simulink model "snap_adc5g_spec_rpi"  (R2019a)
settings: Solver=VariableStepDiscrete  StartTime=0.0  StopTime=10.0  RelTol=1e-3
undefined symbols (not defined in the file): pfb_coeff_gen_calc
libraries: xbsIndex_r4 x13965, casper_library_misc x80, casper_library_delays x43, xps_library x5, xbsReplacements_r4 x2, casper_library_communications x1
(part 7 of 152)

== system snap_adc5g_spec_rpi/fft_wideband_real/fft_direct ==
  sync : Inport
  shift : Inport  Port=2
  in00 : Inport  Port=3
  in01 : Inport  Port=4
  in02 : Inport  Port=5
  in03 : Inport  Port=6
  in10 : Inport  Port=7
  in11 : Inport  Port=8
  in12 : Inport  Port=9
  in13 : Inport  Port=10
  abus : Subsystem  AncestorBlock=casper_library_flow_control/bus_create  mask(bus_create){inputNum=4}
      mask prompts: inputNum "Number of inputs:"
      mask init:
      | bus_create_init(gcb,...
      |     'inputNum', inputNum);
  adebus0_0 : Subsystem  AncestorBlock=casper_library_flow_control/bus_expand  mask(bus_expand){mode=divisions of equal size, outputNum=2, outputWidth=[72 72], outputBinaryPt=[0 0], outputArithmeticType=[0 0], show_format=off, outputToWorkspace=off, variablePrefix=out, outputToModelAsWell=on}
      mask prompts: outputNum "Number of outputs:"; outputWidth "Output width:"; outputBinaryPt "Output binary point position:"; outputArithmeticType "Output arithmetic type (ufix=0, fix=1, bool=2):"; show_format "Print format string?"; outputToWorkspace "Output to workspace?"; variablePrefix "Variable name prefix:"; outputToModelAsWell "Output to model as well?"
      mask help:
      | Expands a 'bus' made using a bus_create or Xilinx
      | concat block.
      | The input will be divided into the specified number
      | of outputs with the specified arithmetic types.
      | Divisions are made from most significant bit.
      mask init: same as snap_adc5g_spec_rpi/ss_adc/ctrl_split
      settings: AttributesFormatString=2 outputs
      mask TypeOptions mode: divisions of equal size | divisions of arbitrary size
      mask Callback mode: bus_expand_callback();
      mask Callback outputWidth: bus_expand_callback();
      mask Callback outputToWorkspace: bus_expand_callback();
  adebus1_0 : Subsystem  AncestorBlock=casper_library_flow_control/bus_expand  mask(bus_expand){mode=divisions of equal size, outputNum=2, outputWidth=[36 36], outputBinaryPt=[0 0], outputArithmeticType=[0 0], show_format=off, outputToWorkspace=off, variablePrefix=out, outputToModelAsWell=on}
      mask prompts: outputNum "Number of outputs:"; outputWidth "Output width:"; outputBinaryPt "Output binary point position:"; outputArithmeticType "Output arithmetic type (ufix=0, fix=1, bool=2):"; show_format "Print format string?"; outputToWorkspace "Output to workspace?"; variablePrefix "Variable name prefix:"; outputToModelAsWell "Output to model as well?"
      mask help:
      | Expands a 'bus' made using a bus_create or Xilinx
      | concat block.
      | The input will be divided into the specified number
      | of outputs with the specified arithmetic types.
      | Divisions are made from most significant bit.
      mask init: same as snap_adc5g_spec_rpi/ss_adc/ctrl_split
      settings: AttributesFormatString=2 outputs
      mask TypeOptions mode: divisions of equal size | divisions of arbitrary size
      mask Callback mode: bus_expand_callback();
      mask Callback outputWidth: bus_expand_callback();
      mask Callback outputToWorkspace: bus_expand_callback();
  adebus1_1 : Subsystem  AncestorBlock=casper_library_flow_control/bus_expand  mask(bus_expand){mode=divisions of equal size, outputNum=2, outputWidth=[36 36], outputBinaryPt=[0 0], outputArithmeticType=[0 0], show_format=off, outputToWorkspace=off, variablePrefix=out, outputToModelAsWell=on}
      mask prompts: outputNum "Number of outputs:"; outputWidth "Output width:"; outputBinaryPt "Output binary point position:"; outputArithmeticType "Output arithmetic type (ufix=0, fix=1, bool=2):"; show_format "Print format string?"; outputToWorkspace "Output to workspace?"; variablePrefix "Variable name prefix:"; outputToModelAsWell "Output to model as well?"
      mask help:
      | Expands a 'bus' made using a bus_create or Xilinx
      | concat block.
      | The input will be divided into the specified number
      | of outputs with the specified arithmetic types.
      | Divisions are made from most significant bit.
      mask init: same as snap_adc5g_spec_rpi/ss_adc/ctrl_split
      settings: AttributesFormatString=2 outputs
      mask TypeOptions mode: divisions of equal size | divisions of arbitrary size
      mask Callback mode: bus_expand_callback();
      mask Callback outputWidth: bus_expand_callback();
      mask Callback outputToWorkspace: bus_expand_callback();
  bbus : Subsystem  AncestorBlock=casper_library_flow_control/bus_create  mask(bus_create){inputNum=4}
      mask prompts: inputNum "Number of inputs:"
      mask init:
      | bus_create_init(gcb,...
      |     'inputNum', inputNum);
  bdebus0_0 : Subsystem  AncestorBlock=casper_library_flow_control/bus_expand  mask(bus_expand){mode=divisions of equal size, outputNum=2, outputWidth=[72 72], outputBinaryPt=[0 0], outputArithmeticType=[0 0], show_format=off, outputToWorkspace=off, variablePrefix=out, outputToModelAsWell=on}
      mask prompts: outputNum "Number of outputs:"; outputWidth "Output width:"; outputBinaryPt "Output binary point position:"; outputArithmeticType "Output arithmetic type (ufix=0, fix=1, bool=2):"; show_format "Print format string?"; outputToWorkspace "Output to workspace?"; variablePrefix "Variable name prefix:"; outputToModelAsWell "Output to model as well?"
      mask help:
      | Expands a 'bus' made using a bus_create or Xilinx
      | concat block.
      | The input will be divided into the specified number
      | of outputs with the specified arithmetic types.
      | Divisions are made from most significant bit.
      mask init: same as snap_adc5g_spec_rpi/ss_adc/ctrl_split
      settings: AttributesFormatString=2 outputs
      mask TypeOptions mode: divisions of equal size | divisions of arbitrary size
      mask Callback mode: bus_expand_callback();
      mask Callback outputWidth: bus_expand_callback();
      mask Callback outputToWorkspace: bus_expand_callback();
  bdebus1_0 : Subsystem  AncestorBlock=casper_library_flow_control/bus_expand  mask(bus_expand){mode=divisions of equal size, outputNum=2, outputWidth=[36 36], outputBinaryPt=[0 0], outputArithmeticType=[0 0], show_format=off, outputToWorkspace=off, variablePrefix=out, outputToModelAsWell=on}
      mask prompts: outputNum "Number of outputs:"; outputWidth "Output width:"; outputBinaryPt "Output binary point position:"; outputArithmeticType "Output arithmetic type (ufix=0, fix=1, bool=2):"; show_format "Print format string?"; outputToWorkspace "Output to workspace?"; variablePrefix "Variable name prefix:"; outputToModelAsWell "Output to model as well?"
      mask help:
      | Expands a 'bus' made using a bus_create or Xilinx
      | concat block.
      | The input will be divided into the specified number
      | of outputs with the specified arithmetic types.
      | Divisions are made from most significant bit.
      mask init: same as snap_adc5g_spec_rpi/ss_adc/ctrl_split
      settings: AttributesFormatString=2 outputs
      mask TypeOptions mode: divisions of equal size | divisions of arbitrary size
      mask Callback mode: bus_expand_callback();
      mask Callback outputWidth: bus_expand_callback();
      mask Callback outputToWorkspace: bus_expand_callback();
  bdebus1_1 : Subsystem  AncestorBlock=casper_library_flow_control/bus_expand  mask(bus_expand){mode=divisions of equal size, outputNum=2, outputWidth=[36 36], outputBinaryPt=[0 0], outputArithmeticType=[0 0], show_format=off, outputToWorkspace=off, variablePrefix=out, outputToModelAsWell=on}
      mask prompts: outputNum "Number of outputs:"; outputWidth "Output width:"; outputBinaryPt "Output binary point position:"; outputArithmeticType "Output arithmetic type (ufix=0, fix=1, bool=2):"; show_format "Print format string?"; outputToWorkspace "Output to workspace?"; variablePrefix "Variable name prefix:"; outputToModelAsWell "Output to model as well?"
      mask help:
      | Expands a 'bus' made using a bus_create or Xilinx
      | concat block.
      | The input will be divided into the specified number
      | of outputs with the specified arithmetic types.
      | Divisions are made from most significant bit.
      mask init: same as snap_adc5g_spec_rpi/ss_adc/ctrl_split
      settings: AttributesFormatString=2 outputs
      mask TypeOptions mode: divisions of equal size | divisions of arbitrary size
      mask Callback mode: bus_expand_callback();
      mask Callback outputWidth: bus_expand_callback();
      mask Callback outputToWorkspace: bus_expand_callback();
  butterfly0_0 : Subsystem  AncestorBlock=casper_library_ffts/butterfly_direct  mask(butterfly_direct){n_inputs=4, biplex=off, FFTSize=13, Coeffs=[ 0 1024 512 1536 256 1280 768 1792 128 1152 640 1664 384 1408 896 1920 64 1088 576 1600 320 1344 832 1856 192 1216 704 1728 448 1472 960 1984 32 1056 544 1568 288 1312 800 1824 160 1184 672 1696 416 1440 928 1952 96 1120 608 1632 352 1376 864 1888 224 1248 736 1760 480 1504 992 2016 16 1040 528 1552 272 1296 784 1808 144 1168 656 1680 400 1424 912 1936 80 1104 592 1616 336 1360 848 1872 208 1232 720 1744 464 1488 976 2000 48 1072 560 1584 304 1328 816 1840 176 1200 688 1712 432 1456 944 1968 112 1136 624 1648 368 1392 880 1904 240 1264 752 1776 496 1520 1008 2032 8 1032 520 1544 264 1288 776 1800 136 1160 648 1672 392 1416 904 1928 72 1096 584 1608 328 1352 840 1864 200 1224 712 1736 456 1480 968 1992 40 1064 552 1576 296 1320 808 1832 168 1192 680 1704 424 1448 936 1960 104 1128 616 1640 360 1384 872 1896 232 1256 744 1768 488 1512 1000 2024 24 1048 536 1560 280 1304 792 1816 152 1176 664 1688 408 1432 920 1944 88 1112 600 1624 344 1368 856 1880 216 1240 728 1752 472 1496 984 2008 56 1080 568 1592 312 1336 824 1848 184 1208 696 1720 440 1464 952 1976 120 1144 632 1656 376 1400 888 1912 248 1272 760 1784 504 1528 1016 2040 4 1028 516 1540 260 1284 772 1796 132 1156 644 1668 388 1412 900 1924 68 1092 580 1604 324 1348 836 1860 196 1220 708 1732 452 1476 964 1988 36 1060 548 1572 292 1316 804 1828 164 1188 676 1700 420 1444 932 1956 100 1124 612 1636 356 1380 868 1892 228 1252 740 1764 484 1508 996 2020 20 1044 532 1556 276 1300 788 1812 148 1172 660 1684 404 1428 916 1940 84 1108 596 1620 340 1364 852 1876 212 1236 724 1748 468 1492 980 2004 52 1076 564 1588 308 1332 820 1844 180 1204 692 1716 436 1460 948 1972 116 1140 628 1652 372 1396 884 1908 244 1268 756 1780 500 1524 1012 2036 12 1036 524 1548 268 1292 780 1804 140 1164 652 1676 396 1420 908 1932 76 1100 588 1612 332 1356 844 1868 204 1228 716 1740 460 1484 972 1996 44 1068 556 1580 300 1324 812 1836 172 1196 684 1708 428 1452 940 1964 108 1132 620 1644 364 1388 876 1900 236 1260 748 1772 492 1516 1004 2028 28 1052 540 1564 284 1308 796 1820 156 1180 668 1692 412 1436 924 1948 92 1116 604 1628 348 1372 860 1884 220 1244 732 1756 476 1500 988 2012 60 1084 572 1596 316 1340 828 1852 188 1212 700 1724 444 1468 956 1980 124 1148 636 1660 380 1404 892 1916 252 1276 764 1788 508 1532 1020 2044 2 1026 514 1538 258 1282 770 1794 130 1154 642 1666 386 1410 898 1922 66 1090 578 1602 322 1346 834 1858 194 1218 706 1730 450 1474 962 1986 34 1058 546 1570 290 1314 802 1826 162 1186 674 1698 418 1442 930 1954 98 1122 610 1634 354 1378 866 1890 226 1250 738 1762 482 1506 994 2018 18 1042 530 1554 274 1298 786 1810 146 1170 658 1682 402 1426 914 1938 82 1106 594 1618 338 1362 850 1874 210 1234 722 1746 466 1490 978 2002 50 1074 562 1586 306 1330 818 1842 178 1202 690 1714 434 1458 946 1970 114 1138 626 1650 370 1394 882 1906 242 1266 754 1778 498 1522 1010 2034 10 1034 522 1546 266 1290 778 1802 138 1162 650 1674 394 1418 906 1930 74 1098 586 1610 330 1354 842 1866 202 1226 714 1738 458 1482 970 1994 42 1066 554 1578 298 1322 810 1834 170 1194 682 1706 426 1450 938 1962 106 1130 618 1642 362 1386 874 1898 234 1258 746 1770 490 1514 1002 2026 26 1050 538 1562 282 1306 794 1818 154 1178 666 1690 410 1434 922 1946 90 1114 602 1626 346 1370 858 1882 218 1242 730 1754 474 1498 986 2010 58 1082 570 1594 314 1338 826 1850 186 1210 698 1722 442 1466 954 1978 122 1146 634 1658 378 1402 890 1914 250 1274 762 1786 506 1530 1018 2042 6 1030 518 1542 262 1286 774 1798 134 1158 646 1670 390 1414 902 1926 70 1094 582 1606 326 1350 838 1862 198 1222 710 1734 454 1478 966 1990 38 1062 550 1574 294 1318 806 1830 166 1190 678 1702 422 1446 934 1958 102 1126 614 1638 358 1382 870 1894 230 1254 742 1766 486 1510 998 2022 22 1046 534 1558 278 1302 790 1814 150 1174 662 1686 406 1430 918 1942 86 1110 598 1622 342 1366 854 1878 214 1238 726 1750 470 1494 982 2006 54 1078 566 1590 310 1334 822 1846 182 1206 694 1718 438 1462 950 1974 118 1142 630 1654 374 1398 886 1910 246 1270 758 1782 502 1526 1014 2038 14 ...(+5134 chars)], StepPeriod=0, coeff_bit_width=18, input_bit_width=18, bin_pt_in=17, downshift=off, async=off, floating_point=off, float_type=single, exp_width=8, frac_width=24, add_latency=1, mult_latency=2, bram_latency=3, conv_latency=1, add_pipe_latency=0, mult_pipe_latency=0, quantization=Round  (unbiased: Even Values), overflow=Wrap, coeffs_bit_limit=9, coeff_sharing=on, coeff_decimation=on, coeff_generation=off, cal_bits=1, n_bits_rotation=25, max_fanout=4, use_hdl=on, use_embedded=off, bitgrowth=off, hardcode_shifts=off, dsp48_adders=off}
      mask prompts: n_inputs "number inputs"; biplex "Used in biplex FFT"; FFTSize "Size of FFT: (2^? pts)"; Coeffs "Coefficients: (0 to 2^(FFTSize-1)-1)"; StepPeriod "Coefficient Step Period: (2^?)"; coeff_bit_width "Coefficient Bit Width"; input_bit_width "Input Bit Width"; bin_pt_in "Input binary point"; async "asynchronous operation"; floating_point "floating point"; float_type "float type"; exp_width "exponent width"; frac_width "fraction width"; add_latency "Add Latency"; mult_latency "Mult Latency"; bram_latency "BRAM Latency"; conv_latency "Convert latency"; add_pipe_latency "Add Pipeline Latency"; mult_pipe_latency "Mult Pipeline Latency"; quantization "Quantization Behavior"; overflow "Overflow Behavior"; coeffs_bit_limit "Number bits above which to store stage's coefficients in BRAM (2^? bits)"; coeff_sharing "BRAM sharing in coeff storage"; coeff_decimation "Store a fraction of coeff factors where useful"; coeff_generation "Generate coeffs with multipliers where useful"; cal_bits "Number calibration locations when generating coeffs (2^?)"; n_bits_rotation "Feedback rotation vector resolution"; max_fanout "Maximum fanout"; use_hdl "Use behavioural HDL for multipliers"; use_embedded "Use embedded multipliers"; bitgrowth "Bit growth instead of shifting"; hardcode_shifts "Hardcode shift schedule"; dsp48_adders "Use DSP48s for adders"
      mask help: FFT internal block.
      mask init:
      | butterfly_direct_init(gcb, ...
      |    'n_inputs', n_inputs, ...
      |    'biplex', biplex, ...
      |    'FFTSize', FFTSize, ...
      |    'Coeffs', Coeffs, ...
      |    'StepPeriod', StepPeriod, ...
      |    'coeff_bit_width', coeff_bit_width, ...
      |    'input_bit_width', input_bit_width, ...
      |    'bin_pt_in', bin_pt_in, ...
      |    'hardcode_shifts', hardcode_shifts, ...
      |    'bitgrowth', bitgrowth, ...
      |    'downshift', downshift, ...
      |    'floating_point', floating_point, ...
      |    'float_type', float_type, ...
      |    'exp_width', exp_width, ...
      |    'frac_width', frac_width, ...   
      |    'async', async, ...
      |    'add_latency', add_latency, ...
      |    'mult_latency', mult_latency, ...
      |    'bram_latency', bram_latency, ...
      |    'conv_latency', conv_latency, ...
      |    'add_pipe_latency', add_pipe_latency, ...
      |    'mult_pipe_latency', mult_pipe_latency, ...        
      |    'quantization', quantization, ...
      |    'overflow', overflow, ...
      |    'coeffs_bit_limit', coeffs_bit_limit, ...    
      |    'coeff_sharing', coeff_sharing, ...
      |    'coeff_decimation', coeff_decimation, ...
      |    'coeff_generation', coeff_generation, ...
      |    'cal_bits', cal_bits, ...
      |    'n_bits_rotation', n_bits_rotation, ...
      |    'max_fanout', max_fanout, ...
      |    'use_hdl', use_hdl, ...
      |    'use_embedded', use_embedded, ...
      |    'dsp48_adders', dsp48_adders);
      settings: AttributesFormatString=twiddle_general
      mask Callback floating_point:
      | onoff = get_param(gcb, 'floating_point');
      | if strcmp(onoff,'on')
      |     enable_fixpt = 'off'
      |     set_param_state(gcb, 'float_type', 'on')
      | 
      |     f_type = get_param(gcb, 'float_type')
      |     if strcmp(f_type,'custom')
      |         set_param_state(gcb, 'exp_width', 'on')
      |         set_param_state(gcb, 'frac_width', 'on')
      |     else
      |         set_param_state(gcb, 'exp_width', 'off')
      |         set_param_state(gcb, 'frac_width', 'off')
      |     end
      | 
      | 
      | else
      |     enable_fixpt = 'on'
      |     set_param_state(gcb, 'float_type', 'off')
      |     set_param_state(gcb, 'exp_width', 'off')
      |     set_param_state(gcb, 'frac_width', 'off')
      | end
      | 
      | set_param_state(gcb, 'input_bit_width', enable_fixpt)
      | set_param_state(gcb, 'bin_pt_in', enable_fixpt)
      | set_param_state(gcb, 'coeff_bit_width', enable_fixpt)
      mask TypeOptions float_type: single | custom
      mask Callback float_type:
      | f_type = get_param(gcb, 'float_type')
      | if strcmp(f_type,'custom')
      |     set_param_state(gcb, 'exp_width', 'on')
      |     set_param_state(gcb, 'frac_width', 'on')
      | else
      |     set_param_state(gcb, 'exp_width', 'off')
      |     set_param_state(gcb, 'frac_width', 'off')
      | end
      mask TypeOptions quantization: Truncate | Round  (unbiased: +/- Inf) | Round  (unbiased: Even Values)
      mask TypeOptions overflow: Wrap | Saturate | Error
      mask Callback use_hdl:
      | % make mutually exclusive with use_embedded.
      | 
      | use_hdl = get_param(gcb, 'use_hdl');
      | if strcmp(use_hdl, 'on'),
      |     set_param_state(gcb, 'use_embedded', 'off');
      | else
      |     set_param_state(gcb, 'use_embedded', 'on');
      | end
      mask Callback use_embedded:
      | % make mutually exclusive with use_hdl.
      | 
      | use_hdl = get_param(gcb, 'use_embedded');
      | if strcmp(use_hdl, 'on'),
      |     set_param_state(gcb, 'use_hdl', 'off');
      | else
      |     set_param_state(gcb, 'use_hdl', 'on');
      | end
      mask Callback hardcode_shifts:
      | hardcode_shifts = get_param(gcb, 'hardcode_shifts');
      | set_param_state(gcb, 'downshift', hardcode_shifts);
      mask Callback dsp48_adders: %fft_callback_dsp48_adders(gcb);
      mask DialogControl ParameterTabVar0 Prompt: Basic
      mask DialogControl ParameterTabVar01 Prompt: Latency
      mask DialogControl ParameterTabVar012 Prompt: Implementation
  butterfly1_0 : Subsystem  AncestorBlock=casper_library_ffts/butterfly_direct  mask(butterfly_direct){n_inputs=2, biplex=off, FFTSize=13, Coeffs=[ 0 2048 1024 3072 512 2560 1536 3584 256 2304 1280 3328 768 2816 1792 3840 128 2176 1152 3200 640 2688 1664 3712 384 2432 1408 3456 896 2944 1920 3968 64 2112 1088 3136 576 2624 1600 3648 320 2368 1344 3392 832 2880 1856 3904 192 2240 1216 3264 704 2752 1728 3776 448 2496 1472 3520 960 3008 1984 4032 32 2080 1056 3104 544 2592 1568 3616 288 2336 1312 3360 800 2848 1824 3872 160 2208 1184 3232 672 2720 1696 3744 416 2464 1440 3488 928 2976 1952 4000 96 2144 1120 3168 608 2656 1632 3680 352 2400 1376 3424 864 2912 1888 3936 224 2272 1248 3296 736 2784 1760 3808 480 2528 1504 3552 992 3040 2016 4064 16 2064 1040 3088 528 2576 1552 3600 272 2320 1296 3344 784 2832 1808 3856 144 2192 1168 3216 656 2704 1680 3728 400 2448 1424 3472 912 2960 1936 3984 80 2128 1104 3152 592 2640 1616 3664 336 2384 1360 3408 848 2896 1872 3920 208 2256 1232 3280 720 2768 1744 3792 464 2512 1488 3536 976 3024 2000 4048 48 2096 1072 3120 560 2608 1584 3632 304 2352 1328 3376 816 2864 1840 3888 176 2224 1200 3248 688 2736 1712 3760 432 2480 1456 3504 944 2992 1968 4016 112 2160 1136 3184 624 2672 1648 3696 368 2416 1392 3440 880 2928 1904 3952 240 2288 1264 3312 752 2800 1776 3824 496 2544 1520 3568 1008 3056 2032 4080 8 2056 1032 3080 520 2568 1544 3592 264 2312 1288 3336 776 2824 1800 3848 136 2184 1160 3208 648 2696 1672 3720 392 2440 1416 3464 904 2952 1928 3976 72 2120 1096 3144 584 2632 1608 3656 328 2376 1352 3400 840 2888 1864 3912 200 2248 1224 3272 712 2760 1736 3784 456 2504 1480 3528 968 3016 1992 4040 40 2088 1064 3112 552 2600 1576 3624 296 2344 1320 3368 808 2856 1832 3880 168 2216 1192 3240 680 2728 1704 3752 424 2472 1448 3496 936 2984 1960 4008 104 2152 1128 3176 616 2664 1640 3688 360 2408 1384 3432 872 2920 1896 3944 232 2280 1256 3304 744 2792 1768 3816 488 2536 1512 3560 1000 3048 2024 4072 24 2072 1048 3096 536 2584 1560 3608 280 2328 1304 3352 792 2840 1816 3864 152 2200 1176 3224 664 2712 1688 3736 408 2456 1432 3480 920 2968 1944 3992 88 2136 1112 3160 600 2648 1624 3672 344 2392 1368 3416 856 2904 1880 3928 216 2264 1240 3288 728 2776 1752 3800 472 2520 1496 3544 984 3032 2008 4056 56 2104 1080 3128 568 2616 1592 3640 312 2360 1336 3384 824 2872 1848 3896 184 2232 1208 3256 696 2744 1720 3768 440 2488 1464 3512 952 3000 1976 4024 120 2168 1144 3192 632 2680 1656 3704 376 2424 1400 3448 888 2936 1912 3960 248 2296 1272 3320 760 2808 1784 3832 504 2552 1528 3576 1016 3064 2040 4088 4 2052 1028 3076 516 2564 1540 3588 260 2308 1284 3332 772 2820 1796 3844 132 2180 1156 3204 644 2692 1668 3716 388 2436 1412 3460 900 2948 1924 3972 68 2116 1092 3140 580 2628 1604 3652 324 2372 1348 3396 836 2884 1860 3908 196 2244 1220 3268 708 2756 1732 3780 452 2500 1476 3524 964 3012 1988 4036 36 2084 1060 3108 548 2596 1572 3620 292 2340 1316 3364 804 2852 1828 3876 164 2212 1188 3236 676 2724 1700 3748 420 2468 1444 3492 932 2980 1956 4004 100 2148 1124 3172 612 2660 1636 3684 356 2404 1380 3428 868 2916 1892 3940 228 2276 1252 3300 740 2788 1764 3812 484 2532 1508 3556 996 3044 2020 4068 20 2068 1044 3092 532 2580 1556 3604 276 2324 1300 3348 788 2836 1812 3860 148 2196 1172 3220 660 2708 1684 3732 404 2452 1428 3476 916 2964 1940 3988 84 2132 1108 3156 596 2644 1620 3668 340 2388 1364 3412 852 2900 1876 3924 212 2260 1236 3284 724 2772 1748 3796 468 2516 1492 3540 980 3028 2004 4052 52 2100 1076 3124 564 2612 1588 3636 308 2356 1332 3380 820 2868 1844 3892 180 2228 1204 3252 692 2740 1716 3764 436 2484 1460 3508 948 2996 1972 4020 116 2164 1140 3188 628 2676 1652 3700 372 2420 1396 3444 884 2932 1908 3956 244 2292 1268 3316 756 2804 1780 3828 500 2548 1524 3572 1012 3060 2036 4084 12 2060 1036 3084 524 2572 1548 3596 268 2316 1292 3340 780 2828 1804 3852 140 2188 1164 3212 652 2700 1676 3724 396 2444 1420 3468 908 2956 1932 3980 76 2124 1100 3148 588 2636 1612 3660 332 2380 1356 3404 844 2892 1868 3916 204 2252 1228 3276 716 2764 1740 3788 460 2508 1484 3532 972 3020 1996 4044 44 2092 1068 3116 556 2604 1580 3628 300 2348 1324 3372 812 2860 ...(+5688 chars)], StepPeriod=0, coeff_bit_width=18, input_bit_width=18, bin_pt_in=17, downshift=off, async=off, floating_point=off, float_type=single, exp_width=8, frac_width=24, add_latency=1, mult_latency=2, bram_latency=3, conv_latency=1, add_pipe_latency=0, mult_pipe_latency=0, quantization=Round  (unbiased: Even Values), overflow=Wrap, coeffs_bit_limit=9, coeff_sharing=on, coeff_decimation=on, coeff_generation=off, cal_bits=1, n_bits_rotation=25, max_fanout=4, use_hdl=on, use_embedded=off, bitgrowth=off, hardcode_shifts=off, dsp48_adders=off}
      mask prompts: n_inputs "number inputs"; biplex "Used in biplex FFT"; FFTSize "Size of FFT: (2^? pts)"; Coeffs "Coefficients: (0 to 2^(FFTSize-1)-1)"; StepPeriod "Coefficient Step Period: (2^?)"; coeff_bit_width "Coefficient Bit Width"; input_bit_width "Input Bit Width"; bin_pt_in "Input binary point"; async "asynchronous operation"; floating_point "floating point"; float_type "float type"; exp_width "exponent width"; frac_width "fraction width"; add_latency "Add Latency"; mult_latency "Mult Latency"; bram_latency "BRAM Latency"; conv_latency "Convert latency"; add_pipe_latency "Add Pipeline Latency"; mult_pipe_latency "Mult Pipeline Latency"; quantization "Quantization Behavior"; overflow "Overflow Behavior"; coeffs_bit_limit "Number bits above which to store stage's coefficients in BRAM (2^? bits)"; coeff_sharing "BRAM sharing in coeff storage"; coeff_decimation "Store a fraction of coeff factors where useful"; coeff_generation "Generate coeffs with multipliers where useful"; cal_bits "Number calibration locations when generating coeffs (2^?)"; n_bits_rotation "Feedback rotation vector resolution"; max_fanout "Maximum fanout"; use_hdl "Use behavioural HDL for multipliers"; use_embedded "Use embedded multipliers"; bitgrowth "Bit growth instead of shifting"; hardcode_shifts "Hardcode shift schedule"; dsp48_adders "Use DSP48s for adders"
      mask help: FFT internal block.
      mask init: same as snap_adc5g_spec_rpi/fft_wideband_real/fft_direct/butterfly0_0
      settings: AttributesFormatString=twiddle_general
      mask Callback floating_point:
      | onoff = get_param(gcb, 'floating_point');
      | if strcmp(onoff,'on')
      |     enable_fixpt = 'off'
      |     set_param_state(gcb, 'float_type', 'on')
      | 
      |     f_type = get_param(gcb, 'float_type')
      |     if strcmp(f_type,'custom')
      |         set_param_state(gcb, 'exp_width', 'on')
      |         set_param_state(gcb, 'frac_width', 'on')
      |     else
      |         set_param_state(gcb, 'exp_width', 'off')
      |         set_param_state(gcb, 'frac_width', 'off')
      |     end
      | 
      | 
      | else
      |     enable_fixpt = 'on'
      |     set_param_state(gcb, 'float_type', 'off')
      |     set_param_state(gcb, 'exp_width', 'off')
      |     set_param_state(gcb, 'frac_width', 'off')
      | end
      | 
      | set_param_state(gcb, 'input_bit_width', enable_fixpt)
      | set_param_state(gcb, 'bin_pt_in', enable_fixpt)
      | set_param_state(gcb, 'coeff_bit_width', enable_fixpt)
      mask TypeOptions float_type: single | custom
      mask Callback float_type:
      | f_type = get_param(gcb, 'float_type')
      | if strcmp(f_type,'custom')
      |     set_param_state(gcb, 'exp_width', 'on')
      |     set_param_state(gcb, 'frac_width', 'on')
      | else
      |     set_param_state(gcb, 'exp_width', 'off')
      |     set_param_state(gcb, 'frac_width', 'off')
      | end
      mask TypeOptions quantization: Truncate | Round  (unbiased: +/- Inf) | Round  (unbiased: Even Values)
      mask TypeOptions overflow: Wrap | Saturate | Error
      mask Callback use_hdl:
      | % make mutually exclusive with use_embedded.
      | 
      | use_hdl = get_param(gcb, 'use_hdl');
      | if strcmp(use_hdl, 'on'),
      |     set_param_state(gcb, 'use_embedded', 'off');
      | else
      |     set_param_state(gcb, 'use_embedded', 'on');
      | end
      mask Callback use_embedded:
      | % make mutually exclusive with use_hdl.
      | 
      | use_hdl = get_param(gcb, 'use_embedded');
      | if strcmp(use_hdl, 'on'),
      |     set_param_state(gcb, 'use_hdl', 'off');
      | else
      |     set_param_state(gcb, 'use_hdl', 'on');
      | end
      mask Callback hardcode_shifts:
      | hardcode_shifts = get_param(gcb, 'hardcode_shifts');
      | set_param_state(gcb, 'downshift', hardcode_shifts);
      mask Callback dsp48_adders: %fft_callback_dsp48_adders(gcb);
      mask DialogControl ParameterTabVar0 Prompt: Basic
      mask DialogControl ParameterTabVar01 Prompt: Latency
      mask DialogControl ParameterTabVar012 Prompt: Implementation
  butterfly1_1 : Subsystem  AncestorBlock=casper_library_ffts/butterfly_direct  mask(butterfly_direct){n_inputs=2, biplex=off, FFTSize=13, Coeffs=[ 1 2049 1025 3073 513 2561 1537 3585 257 2305 1281 3329 769 2817 1793 3841 129 2177 1153 3201 641 2689 1665 3713 385 2433 1409 3457 897 2945 1921 3969 65 2113 1089 3137 577 2625 1601 3649 321 2369 1345 3393 833 2881 1857 3905 193 2241 1217 3265 705 2753 1729 3777 449 2497 1473 3521 961 3009 1985 4033 33 2081 1057 3105 545 2593 1569 3617 289 2337 1313 3361 801 2849 1825 3873 161 2209 1185 3233 673 2721 1697 3745 417 2465 1441 3489 929 2977 1953 4001 97 2145 1121 3169 609 2657 1633 3681 353 2401 1377 3425 865 2913 1889 3937 225 2273 1249 3297 737 2785 1761 3809 481 2529 1505 3553 993 3041 2017 4065 17 2065 1041 3089 529 2577 1553 3601 273 2321 1297 3345 785 2833 1809 3857 145 2193 1169 3217 657 2705 1681 3729 401 2449 1425 3473 913 2961 1937 3985 81 2129 1105 3153 593 2641 1617 3665 337 2385 1361 3409 849 2897 1873 3921 209 2257 1233 3281 721 2769 1745 3793 465 2513 1489 3537 977 3025 2001 4049 49 2097 1073 3121 561 2609 1585 3633 305 2353 1329 3377 817 2865 1841 3889 177 2225 1201 3249 689 2737 1713 3761 433 2481 1457 3505 945 2993 1969 4017 113 2161 1137 3185 625 2673 1649 3697 369 2417 1393 3441 881 2929 1905 3953 241 2289 1265 3313 753 2801 1777 3825 497 2545 1521 3569 1009 3057 2033 4081 9 2057 1033 3081 521 2569 1545 3593 265 2313 1289 3337 777 2825 1801 3849 137 2185 1161 3209 649 2697 1673 3721 393 2441 1417 3465 905 2953 1929 3977 73 2121 1097 3145 585 2633 1609 3657 329 2377 1353 3401 841 2889 1865 3913 201 2249 1225 3273 713 2761 1737 3785 457 2505 1481 3529 969 3017 1993 4041 41 2089 1065 3113 553 2601 1577 3625 297 2345 1321 3369 809 2857 1833 3881 169 2217 1193 3241 681 2729 1705 3753 425 2473 1449 3497 937 2985 1961 4009 105 2153 1129 3177 617 2665 1641 3689 361 2409 1385 3433 873 2921 1897 3945 233 2281 1257 3305 745 2793 1769 3817 489 2537 1513 3561 1001 3049 2025 4073 25 2073 1049 3097 537 2585 1561 3609 281 2329 1305 3353 793 2841 1817 3865 153 2201 1177 3225 665 2713 1689 3737 409 2457 1433 3481 921 2969 1945 3993 89 2137 1113 3161 601 2649 1625 3673 345 2393 1369 3417 857 2905 1881 3929 217 2265 1241 3289 729 2777 1753 3801 473 2521 1497 3545 985 3033 2009 4057 57 2105 1081 3129 569 2617 1593 3641 313 2361 1337 3385 825 2873 1849 3897 185 2233 1209 3257 697 2745 1721 3769 441 2489 1465 3513 953 3001 1977 4025 121 2169 1145 3193 633 2681 1657 3705 377 2425 1401 3449 889 2937 1913 3961 249 2297 1273 3321 761 2809 1785 3833 505 2553 1529 3577 1017 3065 2041 4089 5 2053 1029 3077 517 2565 1541 3589 261 2309 1285 3333 773 2821 1797 3845 133 2181 1157 3205 645 2693 1669 3717 389 2437 1413 3461 901 2949 1925 3973 69 2117 1093 3141 581 2629 1605 3653 325 2373 1349 3397 837 2885 1861 3909 197 2245 1221 3269 709 2757 1733 3781 453 2501 1477 3525 965 3013 1989 4037 37 2085 1061 3109 549 2597 1573 3621 293 2341 1317 3365 805 2853 1829 3877 165 2213 1189 3237 677 2725 1701 3749 421 2469 1445 3493 933 2981 1957 4005 101 2149 1125 3173 613 2661 1637 3685 357 2405 1381 3429 869 2917 1893 3941 229 2277 1253 3301 741 2789 1765 3813 485 2533 1509 3557 997 3045 2021 4069 21 2069 1045 3093 533 2581 1557 3605 277 2325 1301 3349 789 2837 1813 3861 149 2197 1173 3221 661 2709 1685 3733 405 2453 1429 3477 917 2965 1941 3989 85 2133 1109 3157 597 2645 1621 3669 341 2389 1365 3413 853 2901 1877 3925 213 2261 1237 3285 725 2773 1749 3797 469 2517 1493 3541 981 3029 2005 4053 53 2101 1077 3125 565 2613 1589 3637 309 2357 1333 3381 821 2869 1845 3893 181 2229 1205 3253 693 2741 1717 3765 437 2485 1461 3509 949 2997 1973 4021 117 2165 1141 3189 629 2677 1653 3701 373 2421 1397 3445 885 2933 1909 3957 245 2293 1269 3317 757 2805 1781 3829 501 2549 1525 3573 1013 3061 2037 4085 13 2061 1037 3085 525 2573 1549 3597 269 2317 1293 3341 781 2829 1805 3853 141 2189 1165 3213 653 2701 1677 3725 397 2445 1421 3469 909 2957 1933 3981 77 2125 1101 3149 589 2637 1613 3661 333 2381 1357 3405 845 2893 1869 3917 205 2253 1229 3277 717 2765 1741 3789 461 2509 1485 3533 973 3021 1997 4045 45 2093 1069 3117 557 2605 1581 3629 301 2349 1325 3373 813 2861 ...(+5688 chars)], StepPeriod=0, coeff_bit_width=18, input_bit_width=18, bin_pt_in=17, downshift=off, async=off, floating_point=off, float_type=single, exp_width=8, frac_width=24, add_latency=1, mult_latency=2, bram_latency=3, conv_latency=1, add_pipe_latency=0, mult_pipe_latency=0, quantization=Round  (unbiased: Even Values), overflow=Wrap, coeffs_bit_limit=9, coeff_sharing=on, coeff_decimation=on, coeff_generation=off, cal_bits=1, n_bits_rotation=25, max_fanout=4, use_hdl=on, use_embedded=off, bitgrowth=off, hardcode_shifts=off, dsp48_adders=off}
      mask prompts: n_inputs "number inputs"; biplex "Used in biplex FFT"; FFTSize "Size of FFT: (2^? pts)"; Coeffs "Coefficients: (0 to 2^(FFTSize-1)-1)"; StepPeriod "Coefficient Step Period: (2^?)"; coeff_bit_width "Coefficient Bit Width"; input_bit_width "Input Bit Width"; bin_pt_in "Input binary point"; async "asynchronous operation"; floating_point "floating point"; float_type "float type"; exp_width "exponent width"; frac_width "fraction width"; add_latency "Add Latency"; mult_latency "Mult Latency"; bram_latency "BRAM Latency"; conv_latency "Convert latency"; add_pipe_latency "Add Pipeline Latency"; mult_pipe_latency "Mult Pipeline Latency"; quantization "Quantization Behavior"; overflow "Overflow Behavior"; coeffs_bit_limit "Number bits above which to store stage's coefficients in BRAM (2^? bits)"; coeff_sharing "BRAM sharing in coeff storage"; coeff_decimation "Store a fraction of coeff factors where useful"; coeff_generation "Generate coeffs with multipliers where useful"; cal_bits "Number calibration locations when generating coeffs (2^?)"; n_bits_rotation "Feedback rotation vector resolution"; max_fanout "Maximum fanout"; use_hdl "Use behavioural HDL for multipliers"; use_embedded "Use embedded multipliers"; bitgrowth "Bit growth instead of shifting"; hardcode_shifts "Hardcode shift schedule"; dsp48_adders "Use DSP48s for adders"
      mask help: FFT internal block.
      mask init: same as snap_adc5g_spec_rpi/fft_wideband_real/fft_direct/butterfly0_0
      settings: AttributesFormatString=twiddle_general
      mask Callback floating_point:
      | onoff = get_param(gcb, 'floating_point');
      | if strcmp(onoff,'on')
      |     enable_fixpt = 'off'
      |     set_param_state(gcb, 'float_type', 'on')
      | 
      |     f_type = get_param(gcb, 'float_type')
      |     if strcmp(f_type,'custom')
      |         set_param_state(gcb, 'exp_width', 'on')
      |         set_param_state(gcb, 'frac_width', 'on')
      |     else
      |         set_param_state(gcb, 'exp_width', 'off')
      |         set_param_state(gcb, 'frac_width', 'off')
      |     end
      | 
      | 
      | else
      |     enable_fixpt = 'on'
      |     set_param_state(gcb, 'float_type', 'off')
      |     set_param_state(gcb, 'exp_width', 'off')
      |     set_param_state(gcb, 'frac_width', 'off')
      | end
      | 
      | set_param_state(gcb, 'input_bit_width', enable_fixpt)
      | set_param_state(gcb, 'bin_pt_in', enable_fixpt)
      | set_param_state(gcb, 'coeff_bit_width', enable_fixpt)
      mask TypeOptions float_type: single | custom
      mask Callback float_type:
      | f_type = get_param(gcb, 'float_type')
      | if strcmp(f_type,'custom')
      |     set_param_state(gcb, 'exp_width', 'on')
      |     set_param_state(gcb, 'frac_width', 'on')
      | else
      |     set_param_state(gcb, 'exp_width', 'off')
      |     set_param_state(gcb, 'frac_width', 'off')
      | end
      mask TypeOptions quantization: Truncate | Round  (unbiased: +/- Inf) | Round  (unbiased: Even Values)
      mask TypeOptions overflow: Wrap | Saturate | Error
      mask Callback use_hdl:
      | % make mutually exclusive with use_embedded.
      | 
      | use_hdl = get_param(gcb, 'use_hdl');
      | if strcmp(use_hdl, 'on'),
      |     set_param_state(gcb, 'use_embedded', 'off');
      | else
      |     set_param_state(gcb, 'use_embedded', 'on');
      | end
      mask Callback use_embedded:
      | % make mutually exclusive with use_hdl.
      | 
      | use_hdl = get_param(gcb, 'use_embedded');
      | if strcmp(use_hdl, 'on'),
      |     set_param_state(gcb, 'use_hdl', 'off');
      | else
      |     set_param_state(gcb, 'use_hdl', 'on');
      | end
      mask Callback hardcode_shifts:
      | hardcode_shifts = get_param(gcb, 'hardcode_shifts');
      | set_param_state(gcb, 'downshift', hardcode_shifts);
      mask Callback dsp48_adders: %fft_callback_dsp48_adders(gcb);
      mask DialogControl ParameterTabVar0 Prompt: Basic
      mask DialogControl ParameterTabVar01 Prompt: Latency
      mask DialogControl ParameterTabVar012 Prompt: Implementation
  combine : xbsIndex_r4/Logical  logical_function=OR  inputs=2  en=off  latency=2  precision=Full  arith_type=Unsigned  n_bits=16  bin_pt=0  align_bp=on  dbl_ovrd=off  block_type=logical
  of_0 : xbsIndex_r4/Delay  rst=off  infoeditControl=Selection of Reset will increase slice count due to use of real FFs and instead of SRLs  en=off  latency=0  reg_retiming=on  dbl_ovrd=off  block_type=delay
  of_1 : xbsIndex_r4/Concat  num_inputs=2  dbl_ovrd=off  block_type=concat
  of_expand : Subsystem  AncestorBlock=casper_library_flow_control/bus_expand  mask(bus_expand){mode=divisions of equal size, outputNum=2, outputWidth=2, outputBinaryPt=0, outputArithmeticType=0, show_format=off, outputToWorkspace=off, variablePrefix=out, outputToModelAsWell=on}
      mask prompts: outputNum "Number of outputs:"; outputWidth "Output width:"; outputBinaryPt "Output binary point position:"; outputArithmeticType "Output arithmetic type (ufix=0, fix=1, bool=2):"; show_format "Print format string?"; outputToWorkspace "Output to workspace?"; variablePrefix "Variable name prefix:"; outputToModelAsWell "Output to model as well?"
      mask help:
      | Expands a 'bus' made using a bus_create or Xilinx
      | concat block.
      | The input will be divided into the specified number
      | of outputs with the specified arithmetic types.
      | Divisions are made from most significant bit.
      mask init: same as snap_adc5g_spec_rpi/ss_adc/ctrl_split
      settings: AttributesFormatString=2 outputs
      mask TypeOptions mode: divisions of equal size | divisions of arbitrary size
      mask Callback mode: bus_expand_callback();
      mask Callback outputWidth: bus_expand_callback();
      mask Callback outputToWorkspace: bus_expand_callback();
  of_or : xbsIndex_r4/Logical  logical_function=OR  inputs=2  en=off  latency=2  precision=Full  arith_type=Unsigned  n_bits=16  bin_pt=0  align_bp=on  dbl_ovrd=off  block_type=logical
  slice0 : xbsIndex_r4/Slice  nbits=1  boolean_output=on  mode=Lower Bit Location + Width  bit1=0  base1=MSB of Input  bit0=0  base0=LSB of Input  dbl_ovrd=off  block_type=slice
  slice1 : xbsIndex_r4/Slice  nbits=1  boolean_output=on  mode=Lower Bit Location + Width  bit1=0  base1=MSB of Input  bit0=1  base0=LSB of Input  dbl_ovrd=off  block_type=slice
  synct1 : Terminator
  sync_out : Outport
  out00 : Outport  Port=2
  out01 : Outport  Port=3
  out02 : Outport  Port=4
  out03 : Outport  Port=5
  out10 : Outport  Port=6
  out11 : Outport  Port=7
  out12 : Outport  Port=8
  out13 : Outport  Port=9
  of : Outport  Port=10
  wires:
  in00/1 -> abus/1(in1)
  adebus1_0/1(msb_out2) -> out00/1
  in01/1 -> abus/3(in3)
  adebus1_1/1(msb_out2) -> out01/1
  in02/1 -> bbus/1(in1)
  bdebus1_0/1(msb_out2) -> out02/1
  in03/1 -> bbus/3(in3)
  bdebus1_1/1(msb_out2) -> out03/1
  in10/1 -> abus/2(in2)
  adebus1_0/2(lsb_out1) -> out10/1
  in11/1 -> abus/4(in4)
  adebus1_1/2(lsb_out1) -> out11/1
  in12/1 -> bbus/2(in2)
  bdebus1_0/2(lsb_out1) -> out12/1
  in13/1 -> bbus/4(in4)
  bdebus1_1/2(lsb_out1) -> out13/1
  of_or/1 -> of_expand/1(bus_in)
  of_expand/1(msb_out2) -> combine/1
  of_expand/2(lsb_out1) -> combine/2
  combine/1 -> of/1
  shift/1 -> slice0/1, slice1/1
  of_0/1 -> of_or/1
  sync/1 -> butterfly0_0/3(sync_in)
  slice0/1 -> butterfly0_0/4(shift)
  abus/1(bus_out) -> butterfly0_0/1(a)
  bbus/1(bus_out) -> butterfly0_0/2(b)
  butterfly0_0/3(of) -> of_0/1
  butterfly0_0/1(a+bw) -> adebus0_0/1(bus_in)
  butterfly0_0/2(a-bw) -> bdebus0_0/1(bus_in)
  of_1/1 -> of_or/2
  butterfly0_0/4(sync_out) -> butterfly1_0/3(sync_in), butterfly1_1/3(sync_in)
  butterfly1_0/4(sync_out) -> sync_out/1
  slice1/1 -> butterfly1_0/4(shift), butterfly1_1/4(shift)
  adebus0_0/1(msb_out2) -> butterfly1_0/1(a)
  adebus0_0/2(lsb_out1) -> butterfly1_0/2(b)
  butterfly1_0/3(of) -> of_1/1
  butterfly1_1/4(sync_out) -> synct1/1
  bdebus0_0/1(msb_out2) -> butterfly1_1/1(a)
  bdebus0_0/2(lsb_out1) -> butterfly1_1/2(b)
  butterfly1_1/3(of) -> of_1/2
  butterfly1_0/1(a+bw) -> adebus1_0/1(bus_in)
  butterfly1_0/2(a-bw) -> bdebus1_0/1(bus_in)
  butterfly1_1/1(a+bw) -> adebus1_1/1(bus_in)
  butterfly1_1/2(a-bw) -> bdebus1_1/1(bus_in)
